simulink model "Practica3_MSF1_MAT"  (R2024b)
settings: Solver=VariableStepAuto  StartTime=0.0  StopTime=10.0  RelTol=1e-3
libraries: slpidlib x1
settings Model: Creator=ASUS  LastModifiedBy=Angel Torales
settings DataIOCC: SaveOutput=off  SignalLogging=off  DSMLogging=off  ReturnWorkspaceOutputs=off  TimeSaveName=t
settings DebuggingCC: AlgebraicLoopMsg=none  ArtificialAlgebraicLoopMsg=none  MaxConsecutiveZCsMsg=none  OperatingPointInterfaceChecksumMismatchMsg=none

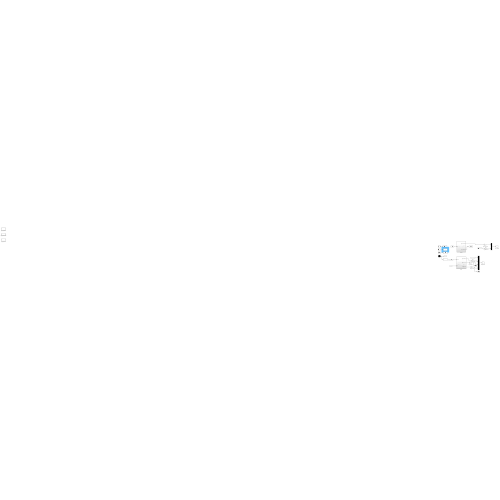
[thumbnail: Simulink's stored preview of the top-level diagram]
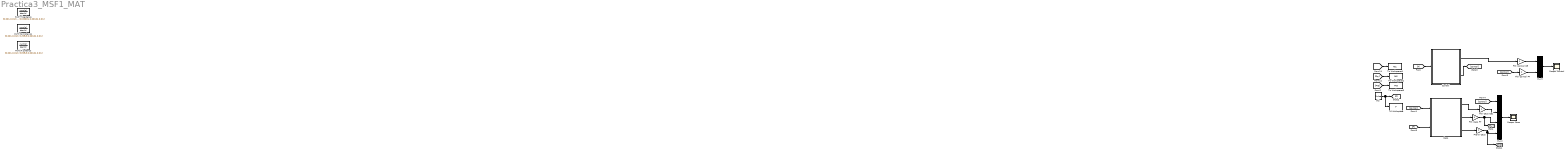
== system Practica3_MSF1_MAT ==
  " Pp(t):Hipertenso" : TransferFcn  Numerator=[0.001,0.01]  Denominator=[0.00001,0.00101,0.01]
  " Pp(t):Hipotenso" : TransferFcn  Numerator=[0.001,0.01]  Denominator=[3.5E-5,0.00101,0.01]
  " Pp(t):Normotenso" : TransferFcn  Numerator=[0.001,0.01]  Denominator=[1.5E-5,0.00101,0.01]
  Caso : Subsystem
  Control : Subsystem
  F(t) : DiscretePulseGenerator  PulseType=Time based  Period=10  PulseWidth=10  PhaseDelay=1
  F(t): Caso CE1 : Gain
  F(t): Caso FT : Gain
  F(t): Control CE : Gain
  F(t): Control FT : Gain
  Mux2 : Mux
  Mux3 : Mux  Inputs=2
  PID(t): Caso : Gain
  Scope: Caso : Scope
  Scope: Control : Scope
  To Workspace : ToWorkspace  VariableName=F  SampleTime=-1
  To Workspace1 : ToWorkspace  VariableName=Fs1  SampleTime=-1
  To Workspace2 : ToWorkspace  VariableName=Fs2  SampleTime=-1
  To Workspace3 : ToWorkspace  VariableName=PID  SampleTime=-1
  wires:
  [F] -> Control/1(F(t))
  Mux2/1 -> Scope: Caso/1
  F(t): Caso FT/1 -> Mux2/3, [Fsy]
  Mux3/1 -> Scope: Control/1
  [control] -> F(t): Control FT/1
  [control] -> To Workspace1/1
  [Fsy] -> To Workspace2/1
  Control/2(F(t): Control FT) -> [control]
  [control] -> Caso/1(Control)
  Caso/2(F(t): Caso FT) -> F(t): Caso FT/1
  [control] -> Mux2/1
  PID(t): Caso/1 -> Mux2/4, [PID]
  Caso/3(PID(t): Caso) -> PID(t): Caso/1
  [PID] -> To Workspace3/1
  F(t)/1 -> To Workspace/1, [F]
  [F] -> Caso/2(F(t))
  F(t): Caso CE1/1 -> Mux2/2
  Caso/1(F(t): Caso CE) -> F(t): Caso CE1/1
  F(t): Control FT/1 -> Mux3/2
  F(t): Control CE/1 -> Mux3/1
  Control/1(F(t): Control CE) -> F(t): Control CE/1

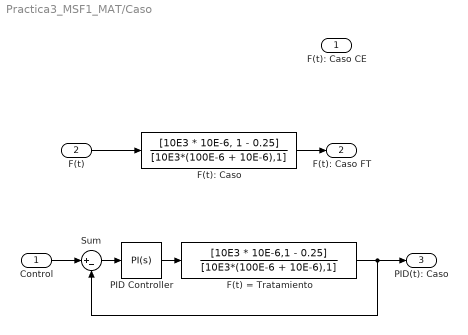
== system Practica3_MSF1_MAT/Caso ==
  Control : Inport
  F(t) : Inport  Port=2
  " F(t) = Tratamiento" : TransferFcn  Numerator=[10E3 * 10E-6,1 - 0.25]  Denominator=[10E3*(100E-6 + 10E-6),1]
  " F(t): Caso" : TransferFcn  Numerator=[10E3 * 10E-6, 1 - 0.25]  Denominator=[10E3*(100E-6 + 10E-6),1]
  PID Controller : slpidlib/PID Controller  Controller=PI  Form=Parallel  TimeDomain=Continuous-time  UseExternalTs=off  SampleTime=-1  IntegratorMethod=Forward Euler  FilterMethod=Forward Euler  ControllerParametersSource=internal  P=0.038181381978369  I=23767.5559547179  UseKiTs=off  D=0.0062671  UseExternalDerivativeSource=off  N=50057.6251  UseFilter=on  TunerSelectOption=Transfer Function Based (PID Tuner App)  InitialConditionSource=internal  InitialConditionForIntegrator=0  InitialConditionForFilter=0  DifferentiatorICPrevScaledInput=0  ExternalReset=none  TrackingMode=off  Kt=1  LimitOutput=off  SatLimitsSource=internal  UpperSaturationLimit=inf  LowerSaturationLimit=-inf  LinearizeAsGain=on  AntiWindupMode=none  Kb=1  LimitIntegrator=off  UpperIntegratorSaturationLimit=inf  LowerIntegratorSaturationLimit=-inf  POutMin=[]  POutMax=[]  IOutMin=[]  IOutMax=[]  DOutMin=[]  DOutMax=[]  NOutMin=[]  NOutMax=[]  SumOutMin=[]  SumOutMax=[]  SaturationOutMin=[]  SaturationOutMax=[]  PParamMin=[]  PParamMax=[]  IParamMin=[]  IParamMax=[]  DParamMin=[]  DParamMax=[]  NParamMin=[]  NParamMax=[]  KbParamMin=[]  KbParamMax=[]  KtParamMin=[]  KtParamMax=[]  KbOutMin=[]  KbOutMax=[]  KtOutMin=[]  KtOutMax=[]  IntegratorOutMin=[]  IntegratorOutMax=[]  FilterOutMin=[]  FilterOutMax=[]  SumI1OutMin=[]  SumI1OutMax=[]  SumI2OutMin=[]  SumI2OutMax=[]  SumI3OutMin=[]  SumI3OutMax=[]  SumI4OutMin=[]  SumI4OutMax=[]  SumDOutMin=[]  SumDOutMax=[]  DifferentiatorOutMin=[]  DifferentiatorOutMax=[]  FilterDiffOutCoefMin=[]  FilterDiffOutCoefMax=[]  ReciprocalOutMin=[]  ReciprocalOutMax=[]  SumDenOutMin=[]  SumDenOutMax=[]  SumNumOutMin=[]  SumNumOutMax=[]  DivideOutMin=[]  DivideOutMax=[]  UdiffTsProdOutMin=[]  UdiffTsProdOutMax=[]  NTsProdOutMin=[]  NTsProdOutMax=[]  UintegralTsProdOutMin=[]  UintegralTsProdOutMax=[]  UngainTsProdOutMin=[]  UngainTsProdOutMax=[]  ClampingZeroOutDataTypeStr=Inherit: Inherit via back propagation  ClampingZeroOutMin=[]  ClampingZeroOutMax=[]  FilterDenConstantOutDataTypeStr=Inherit: Inherit via back propagation  FilterDenConstantOutMin=[]  FilterDenConstantOutMax=[]  PCopyOutDataTypeStr=Inherit: Inherit via back propagation  PCopyOutMin=[]  PCopyOutMax=[]  NCopyOutDataTypeStr=Inherit: Inherit via back propagation  NCopyOutMin=[]  NCopyOutMax=[]  IntegratorContinuousStateAttributes=''  IntegratorStateMustResolveToSignalObject=off  IntegratorRTWStateStorageClass=Auto  FilterContinuousStateAttributes=''  FilterStateMustResolveToSignalObject=off  FilterRTWStateStorageClass=Auto  ParallelPVariant=InternalParameters  IdealPVariant=Disabled  IVariant=InternalParameters  DVariant=Disabled  IntegratorVariant=Continuous  SatVariant=Disabled  AWVariant=Passthrough  PCopyVariant=Disabled  TRVariant=Disabled  FdbkBlocksVariant=Forward  IdealPFdbkVariant=Disabled  SatFdbkVariant=Disabled  DerivativeFilterVariant=Disabled  NVariant=Disabled  NCopyVariant=Disabled_SignalSpec  FilterICVariant=Disabled  IntegratorICVariant=InternalICs  ExternalResetVariant=Disabled  TRSumVariant=Passthrough  SumFdbkVariant=Disabled  SumVariant=Sum_PI  TsampFilterVariant=InternalTs  TsampNgainVariant=Passthrough  TsampIntegralVariant=Disabled_SignalSpec  ExternalSaturationOutDataTypeStr=Inherit: Same as second input  DerivativeSourceVariant=Disabled  PreIntVariant=InternalPreInt
  Sum : Sum  Inputs=|+-
  F(t): Caso CE : Outport
  F(t): Caso FT : Outport  Port=2
  PID(t): Caso : Outport  Port=3
  wires:
  " F(t) = Tratamiento"/1 -> Sum/2, PID(t): Caso/1
  PID Controller/1 -> " F(t) = Tratamiento"/1
  Sum/1 -> PID Controller/1
  Control/1 -> Sum/1
  F(t)/1 -> " F(t): Caso"/1
  " F(t): Caso"/1 -> F(t): Caso FT/1

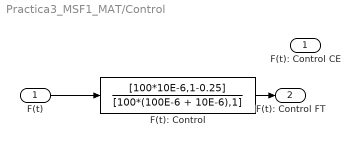
== system Practica3_MSF1_MAT/Control ==
  F(t) : Inport
  " F(t): Control" : TransferFcn  Numerator=[100*10E-6,1-0.25]  Denominator=[100*(100E-6 + 10E-6),1]
  F(t): Control CE : Outport
  F(t): Control FT : Outport  Port=2
  wires:
  F(t)/1 -> " F(t): Control"/1
  " F(t): Control"/1 -> F(t): Control FT/1
